simulink library "sm_wheel_loader_lib"  (R2025a)
settings: Solver=VariableStepAuto  StartTime=0.0  StopTime=10.0  RelTol=1e-3
undefined symbols (not defined in the file): AToTOrificeVector, BiPOrificeVector, boomHEArea, boomREArea, BToTOrificeVector, fluids, GRake, GToothL, GToothR, HMPST, HydFcnParams, logLoad, Position, PToAOrificeVector, PToBOrificeVector, RakeL, RakeR, testInput, Wheel_Loader, X, Y, Z
libraries: sm_lib x694, fl_lib x183, nesl_utility x74, SimscapeFluids_lib x62, sdl_lib x25, cvt_components_lib x25, simulink_extras x5, $bdroot x4, wheel_loader_contact_lib x4, ee_lib x2, SignalEditorBlockLib x1, batteryecm_lib x1
(part 21 of 26)

== system sm_wheel_loader_lib/Wheel Loader Vehicle/Driveline/Driveline/Driveline 3D/Differential F/Stub Shaft R ==
  FDRStubShaft_primary : sm_lib/Body Elements/File Solid  ExtGeomFileName=DiffF_Stub_Shaft_R.STEP  UnitType=FromFile  ExtGeomFileUnits=m  StepReaderType=HEX  ExportConvexHullGeometry=off  InertiaType=Custom  BasedOnType=DensityFromFile  Density=1000  DensityUnits=kg/m^3  Mass=Wheel_Loader.bodyGroups(43).subGroups(1).inertialProperties.mass  MassUnits=kg  CenterOfMass="Wheel_Loader.bodyGroups(43).subGroups(1).inertialProperties.centerOfMass-[0 -0.000000705905842  -0.000000386215069]'"  CenterOfMassUnits=m  MomentsOfInertia=Wheel_Loader.bodyGroups(43).subGroups(1).inertialProperties.momentsOfInertia  MomentsOfInertiaUnits=kg*m^2  ProductsOfInertia=Wheel_Loader.bodyGroups(43).subGroups(1).inertialProperties.productsOfInertia  ProductsOfInertiaUnits=kg*m^2  GraphicType=FromGeometry  MarkerShape=Sphere  MarkerSize=10  GraphicVisPropType=SimpleVisualProperties  GraphicDiffuseColor=Wheel_Loader.bodyGroups(43).subGroups(1).visualProperties.rgb  GraphicOpacity=Wheel_Loader.bodyGroups(43).subGroups(1).visualProperties.opacity  GraphicSpecularColor=[0.5 0.5 0.5 1.0]  GraphicAmbientColor=[0.15 0.15 0.15 1.0]  GraphicEmissiveColor=[0.0 0.0 0.0 1.0]  GraphicShininess=75  DoExposeReferenceFrame=on  SerializedFrames=<Frames/>
  FDRStubShaft_secondary : sm_lib/Body Elements/File Solid  ExtGeomFileName=DiffF_Stub_Shaft_R_Spacer.STEP  UnitType=FromFile  ExtGeomFileUnits=m  StepReaderType=HEX  ExportConvexHullGeometry=off  InertiaType=Custom  BasedOnType=DensityFromFile  Density=1000  DensityUnits=kg/m^3  Mass=Wheel_Loader.bodyGroups(43).subGroups(2).inertialProperties.mass  MassUnits=kg  CenterOfMass="Wheel_Loader.bodyGroups(43).subGroups(2).inertialProperties.centerOfMass-[0 -0.000000705905966  -0.000000386213852]'"  CenterOfMassUnits=m  MomentsOfInertia=Wheel_Loader.bodyGroups(43).subGroups(2).inertialProperties.momentsOfInertia  MomentsOfInertiaUnits=kg*m^2  ProductsOfInertia=Wheel_Loader.bodyGroups(43).subGroups(2).inertialProperties.productsOfInertia  ProductsOfInertiaUnits=kg*m^2  GraphicType=FromGeometry  MarkerShape=Sphere  MarkerSize=10  GraphicVisPropType=SimpleVisualProperties  GraphicDiffuseColor=Wheel_Loader.bodyGroups(43).subGroups(2).visualProperties.rgb  GraphicOpacity=Wheel_Loader.bodyGroups(43).subGroups(2).visualProperties.opacity  GraphicSpecularColor=[0.5 0.5 0.5 1.0]  GraphicAmbientColor=[0.15 0.15 0.15 1.0]  GraphicEmissiveColor=[0.0 0.0 0.0 1.0]  GraphicShininess=75  DoExposeReferenceFrame=on  SerializedFrames=<Frames/>
  RT_FDRStubShaft_RFFDSunGear_Weld : sm_lib/Frames and Transforms/Rigid Transform  RotationMethod=RotationMatrix  FollAlignAxisA=+X  BaseAlignAxisA=+Y  FollAlignAxisB=+Y  BaseAlignAxisB=+Z  RotationStandardAxis=+Z  RotationAngle=0.0  RotationAngleUnits=deg  RotationArbitraryAxis=[0 0 1]  RotationSequenceAxes=FollowerAxes  RotationSequence=XYX  RotationSequenceAngles=[0 0 0]  RotationSequenceAnglesUnits=deg  RotationMatrix=Wheel_Loader.coordSys(66).transform.rotation  Quaternion=[1 0 0 0]  TranslationMethod=Cartesian  TranslationCartesianOffset=Wheel_Loader.coordSys(66).transform.translation  TranslationCartesianOffsetUnits=m  TranslationStandardAxis=+Z  TranslationStandardOffset=0  TranslationStandardOffsetUnits=m  TranslationROffset=0  TranslationROffsetUnits=m  TranslationThetaOffset=0  TranslationThetaOffsetUnits=deg  TranslationZOffset=0  TranslationZOffsetUnits=m
  RT_FDR_StubShaft_Casing : sm_lib/Frames and Transforms/Rigid Transform  RotationMethod=RotationMatrix  FollAlignAxisA=+X  BaseAlignAxisA=+Y  FollAlignAxisB=+Y  BaseAlignAxisB=+Z  RotationStandardAxis=+Z  RotationAngle=0.0  RotationAngleUnits=deg  RotationArbitraryAxis=[0 0 1]  RotationSequenceAxes=FollowerAxes  RotationSequence=XYX  RotationSequenceAngles=[0 0 0]  RotationSequenceAnglesUnits=deg  RotationMatrix=Wheel_Loader.coordSys(49).transform.rotation  Quaternion=[1 0 0 0]  TranslationMethod=Cartesian  TranslationCartesianOffset=Wheel_Loader.coordSys(49).transform.translation  TranslationCartesianOffsetUnits=m  TranslationStandardAxis=+Z  TranslationStandardOffset=0  TranslationStandardOffsetUnits=m  TranslationROffset=0  TranslationROffsetUnits=m  TranslationThetaOffset=0  TranslationThetaOffsetUnits=deg  TranslationZOffset=0  TranslationZOffsetUnits=m
  RT_FDR_StubShaft_SideGear : sm_lib/Frames and Transforms/Rigid Transform  RotationMethod=RotationMatrix  FollAlignAxisA=+X  BaseAlignAxisA=+Y  FollAlignAxisB=+Y  BaseAlignAxisB=+Z  RotationStandardAxis=+Z  RotationAngle=0.0  RotationAngleUnits=deg  RotationArbitraryAxis=[0 0 1]  RotationSequenceAxes=FollowerAxes  RotationSequence=XYX  RotationSequenceAngles=[0 0 0]  RotationSequenceAnglesUnits=deg  RotationMatrix=Wheel_Loader.coordSys(49).transform.rotation  Quaternion=[1 0 0 0]  TranslationMethod=Cartesian  TranslationCartesianOffset=Wheel_Loader.coordSys(49).transform.translation  TranslationCartesianOffsetUnits=m  TranslationStandardAxis=+Z  TranslationStandardOffset=0  TranslationStandardOffsetUnits=m  TranslationROffset=0  TranslationROffsetUnits=m  TranslationThetaOffset=0  TranslationThetaOffsetUnits=deg  TranslationZOffset=0  TranslationZOffsetUnits=m
  RT_FrontAxle_FDRStubShaft : sm_lib/Frames and Transforms/Rigid Transform  RotationMethod=RotationMatrix  FollAlignAxisA=+X  BaseAlignAxisA=+Y  FollAlignAxisB=+Y  BaseAlignAxisB=+Z  RotationStandardAxis=+Z  RotationAngle=0.0  RotationAngleUnits=deg  RotationArbitraryAxis=[0 0 1]  RotationSequenceAxes=FollowerAxes  RotationSequence=XYX  RotationSequenceAngles=[0 0 0]  RotationSequenceAnglesUnits=deg  RotationMatrix=Wheel_Loader.coordSys(49).transform.rotation  Quaternion=[1 0 0 0]  TranslationMethod=Cartesian  TranslationCartesianOffset=Wheel_Loader.coordSys(49).transform.translation  TranslationCartesianOffsetUnits=m  TranslationStandardAxis=+Z  TranslationStandardOffset=0  TranslationStandardOffsetUnits=m  TranslationROffset=0  TranslationROffsetUnits=m  TranslationThetaOffset=0  TranslationThetaOffsetUnits=deg  TranslationZOffset=0  TranslationZOffsetUnits=m
  F3 : PMIOPort  Side=Left
  F1 : PMIOPort  Port=2  Side=Right
  connections:
  RT_FDRStubShaft_RFFDSunGear_Weld/RConn1 -- F3/RConn1
  RT_FDR_StubShaft_SideGear/RConn1 -- F1/RConn1
  RT_FDR_StubShaft_SideGear/LConn1 -- RT_FrontAxle_FDRStubShaft/LConn1 -- FDRStubShaft_secondary/RConn1 -- FDRStubShaft_primary/RConn1 -- RT_FDRStubShaft_RFFDSunGear_Weld/LConn1 -- RT_FDR_StubShaft_Casing/LConn1

== system sm_wheel_loader_lib/Wheel Loader Vehicle/Driveline/Driveline/Driveline 3D/Differential R/Ring Gear ==
  Casing A : sm_lib/Body Elements/File Solid  ExtGeomFileName=DiffR_Casing_A.STEP  UnitType=FromFile  ExtGeomFileUnits=m  StepReaderType=HEX  ExportConvexHullGeometry=off  InertiaType=Custom  BasedOnType=DensityFromFile  Density=1000  DensityUnits=kg/m^3  Mass=Wheel_Loader.bodyGroups(69).subGroups(1).inertialProperties.mass  MassUnits=kg  CenterOfMass=Wheel_Loader.bodyGroups(69).subGroups(1).inertialProperties.centerOfMass  CenterOfMassUnits=m  MomentsOfInertia=Wheel_Loader.bodyGroups(69).subGroups(1).inertialProperties.momentsOfInertia  MomentsOfInertiaUnits=kg*m^2  ProductsOfInertia=Wheel_Loader.bodyGroups(69).subGroups(1).inertialProperties.productsOfInertia  ProductsOfInertiaUnits=kg*m^2  GraphicType=FromGeometry  MarkerShape=Sphere  MarkerSize=10  GraphicVisPropType=SimpleVisualProperties  GraphicDiffuseColor=Wheel_Loader.bodyGroups(69).subGroups(1).visualProperties.rgb  GraphicOpacity=diffR_casing_opc  GraphicSpecularColor=[0.5 0.5 0.5 1.0]  GraphicAmbientColor=[0.15 0.15 0.15 1.0]  GraphicEmissiveColor=[0.0 0.0 0.0 1.0]  GraphicShininess=75  DoExposeReferenceFrame=on  SerializedFrames=<Frames/>
  Casing B : sm_lib/Body Elements/File Solid  ExtGeomFileName=DiffR_Casing_B.STEP  UnitType=FromFile  ExtGeomFileUnits=m  StepReaderType=HEX  ExportConvexHullGeometry=off  InertiaType=Custom  BasedOnType=DensityFromFile  Density=1000  DensityUnits=kg/m^3  Mass=Wheel_Loader.bodyGroups(69).subGroups(2).inertialProperties.mass  MassUnits=kg  CenterOfMass=Wheel_Loader.bodyGroups(69).subGroups(2).inertialProperties.centerOfMass  CenterOfMassUnits=m  MomentsOfInertia=Wheel_Loader.bodyGroups(69).subGroups(2).inertialProperties.momentsOfInertia  MomentsOfInertiaUnits=kg*m^2  ProductsOfInertia=Wheel_Loader.bodyGroups(69).subGroups(2).inertialProperties.productsOfInertia  ProductsOfInertiaUnits=kg*m^2  GraphicType=FromGeometry  MarkerShape=Sphere  MarkerSize=10  GraphicVisPropType=SimpleVisualProperties  GraphicDiffuseColor=Wheel_Loader.bodyGroups(69).subGroups(2).visualProperties.rgb  GraphicOpacity=diffR_casing_opc  GraphicSpecularColor=[0.5 0.5 0.5 1.0]  GraphicAmbientColor=[0.15 0.15 0.15 1.0]  GraphicEmissiveColor=[0.0 0.0 0.0 1.0]  GraphicShininess=75  DoExposeReferenceFrame=on  SerializedFrames=<Frames/>
  RT_RDL_StubShaft_Casing : sm_lib/Frames and Transforms/Rigid Transform  RotationMethod=RotationMatrix  FollAlignAxisA=+X  BaseAlignAxisA=+Y  FollAlignAxisB=+Y  BaseAlignAxisB=+Z  RotationStandardAxis=+Z  RotationAngle=0.0  RotationAngleUnits=deg  RotationArbitraryAxis=[0 0 1]  RotationSequenceAxes=FollowerAxes  RotationSequence=XYX  RotationSequenceAngles=[0 0 0]  RotationSequenceAnglesUnits=deg  RotationMatrix=Wheel_Loader.coordSys(48).transform.rotation  Quaternion=[1 0 0 0]  TranslationMethod=Cartesian  TranslationCartesianOffset=Wheel_Loader.coordSys(48).transform.translation  TranslationCartesianOffsetUnits=m  TranslationStandardAxis=+Z  TranslationStandardOffset=0  TranslationStandardOffsetUnits=m  TranslationROffset=0  TranslationROffsetUnits=m  TranslationThetaOffset=0  TranslationThetaOffsetUnits=deg  TranslationZOffset=0  TranslationZOffsetUnits=m
  RT_RD_Pinion_Ring_BGC : sm_lib/Frames and Transforms/Rigid Transform  RotationMethod=RotationMatrix  FollAlignAxisA=+X  BaseAlignAxisA=+Y  FollAlignAxisB=+Y  BaseAlignAxisB=+Z  RotationStandardAxis=+Z  RotationAngle=0.0  RotationAngleUnits=deg  RotationArbitraryAxis=[0 0 1]  RotationSequenceAxes=FollowerAxes  RotationSequence=XYX  RotationSequenceAngles=[0 0 0]  RotationSequenceAnglesUnits=deg  RotationMatrix=Wheel_Loader.coordSys(47).transform.rotation  Quaternion=[1 0 0 0]  TranslationMethod=Cartesian  TranslationCartesianOffset=Wheel_Loader.coordSys(47).transform.translation  TranslationCartesianOffsetUnits=m  TranslationStandardAxis=+Z  TranslationStandardOffset=0  TranslationStandardOffsetUnits=m  TranslationROffset=0  TranslationROffsetUnits=m  TranslationThetaOffset=0  TranslationThetaOffsetUnits=deg  TranslationZOffset=0  TranslationZOffsetUnits=m
  Ring Gear : sm_lib/Body Elements/File Solid  ExtGeomFileName=DiffR_Ring_Gear.STEP  UnitType=FromFile  ExtGeomFileUnits=m  StepReaderType=HEX  ExportConvexHullGeometry=off  InertiaType=Custom  BasedOnType=DensityFromFile  Density=1000  DensityUnits=kg/m^3  Mass=Wheel_Loader.bodyGroups(65).subGroups(1).inertialProperties.mass  MassUnits=kg  CenterOfMass=Wheel_Loader.bodyGroups(65).subGroups(1).inertialProperties.centerOfMass  CenterOfMassUnits=m  MomentsOfInertia=Wheel_Loader.bodyGroups(65).subGroups(1).inertialProperties.momentsOfInertia  MomentsOfInertiaUnits=kg*m^2  ProductsOfInertia=Wheel_Loader.bodyGroups(65).subGroups(1).inertialProperties.productsOfInertia  ProductsOfInertiaUnits=kg*m^2  GraphicType=FromGeometry  MarkerShape=Sphere  MarkerSize=10  GraphicVisPropType=SimpleVisualProperties  GraphicDiffuseColor=Wheel_Loader.bodyGroups(65).subGroups(1).visualProperties.rgb  GraphicOpacity=Wheel_Loader.bodyGroups(65).subGroups(1).visualProperties.opacity  GraphicSpecularColor=[0.5 0.5 0.5 1.0]  GraphicAmbientColor=[0.15 0.15 0.15 1.0]  GraphicEmissiveColor=[0.0 0.0 0.0 1.0]  GraphicShininess=75  DoExposeReferenceFrame=on  SerializedFrames=<Frames/>
  Transform CG : sm_lib/Frames and Transforms/Rigid Transform  RotationMethod=None  FollAlignAxisA=+X  BaseAlignAxisA=+Y  FollAlignAxisB=+Y  BaseAlignAxisB=+Z  RotationStandardAxis=+Z  RotationAngle=0.0  RotationAngleUnits=deg  RotationArbitraryAxis=[0 0 1]  RotationSequenceAxes=FollowerAxes  RotationSequence=XYX  RotationSequenceAngles=[0 0 0]  RotationSequenceAnglesUnits=deg  RotationMatrix=[1 0 0; 0 1 0; 0 0 1]  Quaternion=[1 0 0 0]  TranslationMethod=Cartesian  TranslationCartesianOffset=[0 -0.000000002038373 0.000000042999574]  TranslationCartesianOffsetUnits=m  TranslationStandardAxis=+Z  TranslationStandardOffset=0  TranslationStandardOffsetUnits=m  TranslationROffset=0  TranslationROffsetUnits=m  TranslationThetaOffset=0  TranslationThetaOffsetUnits=deg  TranslationZOffset=0  TranslationZOffsetUnits=m
  Transform Side Gear L : sm_lib/Frames and Transforms/Rigid Transform  RotationMethod=StandardAxis  FollAlignAxisA=+X  BaseAlignAxisA=+Y  FollAlignAxisB=+Y  BaseAlignAxisB=+Z  RotationStandardAxis=+Y  RotationAngle=-90  RotationAngleUnits=deg  RotationArbitraryAxis=[0 0 1]  RotationSequenceAxes=FollowerAxes  RotationSequence=XYX  RotationSequenceAngles=[0 0 0]  RotationSequenceAnglesUnits=deg  RotationMatrix=[1 0 0; 0 1 0; 0 0 1]  Quaternion=[1 0 0 0]  TranslationMethod=Cartesian  TranslationCartesianOffset=[0.056 0 0.0896 ]/2  TranslationCartesianOffsetUnits=m  TranslationStandardAxis=+Z  TranslationStandardOffset=0  TranslationStandardOffsetUnits=m  TranslationROffset=0  TranslationROffsetUnits=m  TranslationThetaOffset=0  TranslationThetaOffsetUnits=deg  TranslationZOffset=0  TranslationZOffsetUnits=m
  Transform Spider Gear 2 : sm_lib/Frames and Transforms/Rigid Transform  RotationMethod=StandardAxis  FollAlignAxisA=+X  BaseAlignAxisA=+Y  FollAlignAxisB=+Y  BaseAlignAxisB=+Z  RotationStandardAxis=+Y  RotationAngle=-90  RotationAngleUnits=deg  RotationArbitraryAxis=[0 0 1]  RotationSequenceAxes=FollowerAxes  RotationSequence=XYX  RotationSequenceAngles=[0 0 0]  RotationSequenceAnglesUnits=deg  RotationMatrix=[1 0 0; 0 1 0; 0 0 1]  Quaternion=[1 0 0 0]  TranslationMethod=Cartesian  TranslationCartesianOffset=[0.0896 0 0.056]/2  TranslationCartesianOffsetUnits=m  TranslationStandardAxis=+Z  TranslationStandardOffset=0  TranslationStandardOffsetUnits=m  TranslationROffset=0  TranslationROffsetUnits=m  TranslationThetaOffset=0  TranslationThetaOffsetUnits=deg  TranslationZOffset=0  TranslationZOffsetUnits=m
  Pin : PMIOPort  Side=Left
  SGR : PMIOPort  Port=2  Side=Right
  connections:
  RT_RD_Pinion_Ring_BGC/LConn1 -- Ring Gear/RConn1 -- RT_RDL_StubShaft_Casing/LConn1 -- Transform CG/LConn1
  RT_RDL_StubShaft_Casing/RConn1 -- Transform Spider Gear 2/LConn1
  RT_RD_Pinion_Ring_BGC/RConn1 -- Pin/RConn1
  Transform CG/RConn1 -- Casing A/RConn1 -- Casing B/RConn1
  Transform Spider Gear 2/RConn1 -- Transform Side Gear L/LConn1
  SGR/RConn1 -- Transform Side Gear L/RConn1

== system sm_wheel_loader_lib/Wheel Loader Vehicle/Driveline/Driveline/Driveline 3D/Differential R/Side Gear L ==
  RT_RDL_StubShaft_SideGear : sm_lib/Frames and Transforms/Rigid Transform  RotationMethod=RotationMatrix  FollAlignAxisA=+X  BaseAlignAxisA=+Y  FollAlignAxisB=+Y  BaseAlignAxisB=+Z  RotationStandardAxis=+Z  RotationAngle=0.0  RotationAngleUnits=deg  RotationArbitraryAxis=[0 0 1]  RotationSequenceAxes=FollowerAxes  RotationSequence=XYX  RotationSequenceAngles=[0 0 0]  RotationSequenceAnglesUnits=deg  RotationMatrix=Wheel_Loader.coordSys(48).transform.rotation  Quaternion=[1 0 0 0]  TranslationMethod=Cartesian  TranslationCartesianOffset=Wheel_Loader.coordSys(48).transform.translation  TranslationCartesianOffsetUnits=m  TranslationStandardAxis=+Z  TranslationStandardOffset=0  TranslationStandardOffsetUnits=m  TranslationROffset=0  TranslationROffsetUnits=m  TranslationThetaOffset=0  TranslationThetaOffsetUnits=deg  TranslationZOffset=0  TranslationZOffsetUnits=m
  RT_RDSpiderGear1_RDLSideGear_BGC : sm_lib/Frames and Transforms/Rigid Transform  RotationMethod=RotationMatrix  FollAlignAxisA=+X  BaseAlignAxisA=+Y  FollAlignAxisB=+Y  BaseAlignAxisB=+Z  RotationStandardAxis=+Z  RotationAngle=0.0  RotationAngleUnits=deg  RotationArbitraryAxis=[0 0 1]  RotationSequenceAxes=FollowerAxes  RotationSequence=XYX  RotationSequenceAngles=[0 0 0]  RotationSequenceAnglesUnits=deg  RotationMatrix=Wheel_Loader.coordSys(48).transform.rotation  Quaternion=[1 0 0 0]  TranslationMethod=Cartesian  TranslationCartesianOffset=Wheel_Loader.coordSys(48).transform.translation  TranslationCartesianOffsetUnits=m  TranslationStandardAxis=+Z  TranslationStandardOffset=0  TranslationStandardOffsetUnits=m  TranslationROffset=0  TranslationROffsetUnits=m  TranslationThetaOffset=0  TranslationThetaOffsetUnits=deg  TranslationZOffset=0  TranslationZOffsetUnits=m
  RT_RDSpiderGear2_RDLSideGear_BGC : sm_lib/Frames and Transforms/Rigid Transform  RotationMethod=RotationMatrix  FollAlignAxisA=+X  BaseAlignAxisA=+Y  FollAlignAxisB=+Y  BaseAlignAxisB=+Z  RotationStandardAxis=+Z  RotationAngle=0.0  RotationAngleUnits=deg  RotationArbitraryAxis=[0 0 1]  RotationSequenceAxes=FollowerAxes  RotationSequence=XYX  RotationSequenceAngles=[0 0 0]  RotationSequenceAnglesUnits=deg  RotationMatrix=Wheel_Loader.coordSys(48).transform.rotation  Quaternion=[1 0 0 0]  TranslationMethod=Cartesian  TranslationCartesianOffset=Wheel_Loader.coordSys(48).transform.translation  TranslationCartesianOffsetUnits=m  TranslationStandardAxis=+Z  TranslationStandardOffset=0  TranslationStandardOffsetUnits=m  TranslationROffset=0  TranslationROffsetUnits=m  TranslationThetaOffset=0  TranslationThetaOffsetUnits=deg  TranslationZOffset=0  TranslationZOffsetUnits=m
  Side Gear L : sm_lib/Body Elements/File Solid  ExtGeomFileName=DiffR_Side_Gear_L.STEP  UnitType=FromFile  ExtGeomFileUnits=m  StepReaderType=HEX  ExportConvexHullGeometry=off  InertiaType=Custom  BasedOnType=DensityFromFile  Density=1000  DensityUnits=kg/m^3  Mass=Wheel_Loader.bodyGroups(57).subGroups(1).inertialProperties.mass  MassUnits=kg  CenterOfMass=Wheel_Loader.bodyGroups(57).subGroups(1).inertialProperties.centerOfMass  CenterOfMassUnits=m  MomentsOfInertia=Wheel_Loader.bodyGroups(57).subGroups(1).inertialProperties.momentsOfInertia  MomentsOfInertiaUnits=kg*m^2  ProductsOfInertia=Wheel_Loader.bodyGroups(57).subGroups(1).inertialProperties.productsOfInertia  ProductsOfInertiaUnits=kg*m^2  GraphicType=FromGeometry  MarkerShape=Sphere  MarkerSize=10  GraphicVisPropType=SimpleVisualProperties  GraphicDiffuseColor=Wheel_Loader.bodyGroups(57).subGroups(1).visualProperties.rgb  GraphicOpacity=Wheel_Loader.bodyGroups(57).subGroups(1).visualProperties.opacity  GraphicSpecularColor=[0.5 0.5 0.5 1.0]  GraphicAmbientColor=[0.15 0.15 0.15 1.0]  GraphicEmissiveColor=[0.0 0.0 0.0 1.0]  GraphicShininess=75  DoExposeReferenceFrame=on  SerializedFrames=<Frames/>
  B : PMIOPort  Side=Left
  F : PMIOPort  Port=2  Side=Right
  connections:
  B/RConn1 -- RT_RDL_StubShaft_SideGear/RConn1 -- F/RConn1
  RT_RDSpiderGear2_RDLSideGear_BGC/LConn1 -- RT_RDSpiderGear1_RDLSideGear_BGC/LConn1 -- Side Gear L/RConn1 -- RT_RDL_StubShaft_SideGear/LConn1

== system sm_wheel_loader_lib/Wheel Loader Vehicle/Driveline/Driveline/Driveline 3D/Differential R/Side Gear R ==
  RT_RDSpiderGear1toRDRSideGear_BGC : sm_lib/Frames and Transforms/Rigid Transform  RotationMethod=RotationMatrix  FollAlignAxisA=+X  BaseAlignAxisA=+Y  FollAlignAxisB=+Y  BaseAlignAxisB=+Z  RotationStandardAxis=+Z  RotationAngle=0.0  RotationAngleUnits=deg  RotationArbitraryAxis=[0 0 1]  RotationSequenceAxes=FollowerAxes  RotationSequence=XYX  RotationSequenceAngles=[0 0 0]  RotationSequenceAnglesUnits=deg  RotationMatrix=Wheel_Loader.coordSys(52).transform.rotation  Quaternion=[1 0 0 0]  TranslationMethod=Cartesian  TranslationCartesianOffset=Wheel_Loader.coordSys(52).transform.translation  TranslationCartesianOffsetUnits=m  TranslationStandardAxis=+Z  TranslationStandardOffset=0  TranslationStandardOffsetUnits=m  TranslationROffset=0  TranslationROffsetUnits=m  TranslationThetaOffset=0  TranslationThetaOffsetUnits=deg  TranslationZOffset=0  TranslationZOffsetUnits=m
  Side Gear R : sm_lib/Body Elements/File Solid  ExtGeomFileName=DiffR_Side_Gear_R.STEP  UnitType=FromFile  ExtGeomFileUnits=m  StepReaderType=HEX  ExportConvexHullGeometry=off  InertiaType=Custom  BasedOnType=DensityFromFile  Density=1000  DensityUnits=kg/m^3  Mass=Wheel_Loader.bodyGroups(56).subGroups(1).inertialProperties.mass  MassUnits=kg  CenterOfMass=Wheel_Loader.bodyGroups(56).subGroups(1).inertialProperties.centerOfMass  CenterOfMassUnits=m  MomentsOfInertia=Wheel_Loader.bodyGroups(56).subGroups(1).inertialProperties.momentsOfInertia  MomentsOfInertiaUnits=kg*m^2  ProductsOfInertia=Wheel_Loader.bodyGroups(56).subGroups(1).inertialProperties.productsOfInertia  ProductsOfInertiaUnits=kg*m^2  GraphicType=FromGeometry  MarkerShape=Sphere  MarkerSize=10  GraphicVisPropType=SimpleVisualProperties  GraphicDiffuseColor=Wheel_Loader.bodyGroups(56).subGroups(1).visualProperties.rgb  GraphicOpacity=Wheel_Loader.bodyGroups(56).subGroups(1).visualProperties.opacity  GraphicSpecularColor=[0.5 0.5 0.5 1.0]  GraphicAmbientColor=[0.15 0.15 0.15 1.0]  GraphicEmissiveColor=[0.0 0.0 0.0 1.0]  GraphicShininess=75  DoExposeReferenceFrame=on  SerializedFrames=<Frames/>
  B : PMIOPort  Side=Left
  F : PMIOPort  Port=2  Side=Right
  connections:
  Side Gear R/RConn1 -- RT_RDSpiderGear1toRDRSideGear_BGC/LConn1
  B/RConn1 -- RT_RDSpiderGear1toRDRSideGear_BGC/RConn1 -- F/RConn1

== system sm_wheel_loader_lib/Wheel Loader Vehicle/Driveline/Driveline/Driveline 3D/Differential R/Spider Gear 1 ==
  Gear : sm_lib/Body Elements/File Solid  ExtGeomFileName=DiffR_Spider_Gear1.STEP  UnitType=FromFile  ExtGeomFileUnits=m  StepReaderType=HEX  ExportConvexHullGeometry=off  InertiaType=Custom  BasedOnType=DensityFromFile  Density=1000  DensityUnits=kg/m^3  Mass=Wheel_Loader.bodyGroups(61).subGroups(1).inertialProperties.mass  MassUnits=kg  CenterOfMass=Wheel_Loader.bodyGroups(61).subGroups(1).inertialProperties.centerOfMass  CenterOfMassUnits=m  MomentsOfInertia=Wheel_Loader.bodyGroups(61).subGroups(1).inertialProperties.momentsOfInertia  MomentsOfInertiaUnits=kg*m^2  ProductsOfInertia=Wheel_Loader.bodyGroups(61).subGroups(1).inertialProperties.productsOfInertia  ProductsOfInertiaUnits=kg*m^2  GraphicType=FromGeometry  MarkerShape=Sphere  MarkerSize=10  GraphicVisPropType=SimpleVisualProperties  GraphicDiffuseColor=Wheel_Loader.bodyGroups(61).subGroups(1).visualProperties.rgb  GraphicOpacity=Wheel_Loader.bodyGroups(61).subGroups(1).visualProperties.opacity  GraphicSpecularColor=[0.5 0.5 0.5 1.0]  GraphicAmbientColor=[0.15 0.15 0.15 1.0]  GraphicEmissiveColor=[0.0 0.0 0.0 1.0]  GraphicShininess=75  DoExposeReferenceFrame=on  SerializedFrames=<Frames/>
  RT_RDSpiderGear1_RDLSideGear_BGC : sm_lib/Frames and Transforms/Rigid Transform  RotationMethod=RotationMatrix  FollAlignAxisA=+X  BaseAlignAxisA=+Y  FollAlignAxisB=+Y  BaseAlignAxisB=+Z  RotationStandardAxis=+Z  RotationAngle=0.0  RotationAngleUnits=deg  RotationArbitraryAxis=[0 0 1]  RotationSequenceAxes=FollowerAxes  RotationSequence=XYX  RotationSequenceAngles=[0 0 0]  RotationSequenceAnglesUnits=deg  RotationMatrix=Wheel_Loader.coordSys(54).transform.rotation  Quaternion=[1 0 0 0]  TranslationMethod=Cartesian  TranslationCartesianOffset=Wheel_Loader.coordSys(54).transform.translation  TranslationCartesianOffsetUnits=m  TranslationStandardAxis=+Z  TranslationStandardOffset=0  TranslationStandardOffsetUnits=m  TranslationROffset=0  TranslationROffsetUnits=m  TranslationThetaOffset=0  TranslationThetaOffsetUnits=deg  TranslationZOffset=0  TranslationZOffsetUnits=m
  RT_RDSpiderGear1toRDRSideGear_BGC : sm_lib/Frames and Transforms/Rigid Transform  RotationMethod=RotationMatrix  FollAlignAxisA=+X  BaseAlignAxisA=+Y  FollAlignAxisB=+Y  BaseAlignAxisB=+Z  RotationStandardAxis=+Z  RotationAngle=0.0  RotationAngleUnits=deg  RotationArbitraryAxis=[0 0 1]  RotationSequenceAxes=FollowerAxes  RotationSequence=XYX  RotationSequenceAngles=[0 0 0]  RotationSequenceAnglesUnits=deg  RotationMatrix=Wheel_Loader.coordSys(54).transform.rotation  Quaternion=[1 0 0 0]  TranslationMethod=Cartesian  TranslationCartesianOffset=Wheel_Loader.coordSys(54).transform.translation  TranslationCartesianOffsetUnits=m  TranslationStandardAxis=+Z  TranslationStandardOffset=0  TranslationStandardOffsetUnits=m  TranslationROffset=0  TranslationROffsetUnits=m  TranslationThetaOffset=0  TranslationThetaOffsetUnits=deg  TranslationZOffset=0  TranslationZOffsetUnits=m
  RT_RD_Casing_SpiderGear1 : sm_lib/Frames and Transforms/Rigid Transform  RotationMethod=RotationMatrix  FollAlignAxisA=+X  BaseAlignAxisA=+Y  FollAlignAxisB=+Y  BaseAlignAxisB=+Z  RotationStandardAxis=+Z  RotationAngle=0.0  RotationAngleUnits=deg  RotationArbitraryAxis=[0 0 1]  RotationSequenceAxes=FollowerAxes  RotationSequence=XYX  RotationSequenceAngles=[0 0 0]  RotationSequenceAnglesUnits=deg  RotationMatrix=Wheel_Loader.coordSys(54).transform.rotation  Quaternion=[1 0 0 0]  TranslationMethod=Cartesian  TranslationCartesianOffset=Wheel_Loader.coordSys(54).transform.translation  TranslationCartesianOffsetUnits=m  TranslationStandardAxis=+Z  TranslationStandardOffset=0  TranslationStandardOffsetUnits=m  TranslationROffset=0  TranslationROffsetUnits=m  TranslationThetaOffset=0  TranslationThetaOffsetUnits=deg  TranslationZOffset=0  TranslationZOffsetUnits=m
  Shaft : sm_lib/Body Elements/File Solid  ExtGeomFileName=DiffR_Spider_Gear1_Shaft.STEP  UnitType=FromFile  ExtGeomFileUnits=m  StepReaderType=HEX  ExportConvexHullGeometry=off  InertiaType=Custom  BasedOnType=DensityFromFile  Density=1000  DensityUnits=kg/m^3  Mass=Wheel_Loader.bodyGroups(61).subGroups(2).inertialProperties.mass  MassUnits=kg  CenterOfMass=Wheel_Loader.bodyGroups(61).subGroups(2).inertialProperties.centerOfMass  CenterOfMassUnits=m  MomentsOfInertia=Wheel_Loader.bodyGroups(61).subGroups(2).inertialProperties.momentsOfInertia  MomentsOfInertiaUnits=kg*m^2  ProductsOfInertia=Wheel_Loader.bodyGroups(61).subGroups(2).inertialProperties.productsOfInertia  ProductsOfInertiaUnits=kg*m^2  GraphicType=FromGeometry  MarkerShape=Sphere  MarkerSize=10  GraphicVisPropType=SimpleVisualProperties  GraphicDiffuseColor=Wheel_Loader.bodyGroups(61).subGroups(2).visualProperties.rgb  GraphicOpacity=Wheel_Loader.bodyGroups(61).subGroups(2).visualProperties.opacity  GraphicSpecularColor=[0.5 0.5 0.5 1.0]  GraphicAmbientColor=[0.15 0.15 0.15 1.0]  GraphicEmissiveColor=[0.0 0.0 0.0 1.0]  GraphicShininess=75  DoExposeReferenceFrame=on  SerializedFrames=<Frames/>
  B : PMIOPort  Side=Left
  F : PMIOPort  Port=2  Side=Right
  connections:
  B/RConn1 -- RT_RD_Casing_SpiderGear1/RConn1 -- F/RConn1
  RT_RD_Casing_SpiderGear1/LConn1 -- Shaft/RConn1 -- Gear/RConn1 -- RT_RDSpiderGear1toRDRSideGear_BGC/LConn1 -- RT_RDSpiderGear1_RDLSideGear_BGC/LConn1

== system sm_wheel_loader_lib/Wheel Loader Vehicle/Driveline/Driveline/Driveline 3D/Differential R/Spider Gear 2 ==
  Gear : sm_lib/Body Elements/File Solid  ExtGeomFileName=DiffR_Spider_Gear2.STEP  UnitType=FromFile  ExtGeomFileUnits=m  StepReaderType=HEX  ExportConvexHullGeometry=off  InertiaType=Custom  BasedOnType=DensityFromFile  Density=1000  DensityUnits=kg/m^3  Mass=Wheel_Loader.bodyGroups(67).subGroups(1).inertialProperties.mass  MassUnits=kg  CenterOfMass=Wheel_Loader.bodyGroups(67).subGroups(1).inertialProperties.centerOfMass  CenterOfMassUnits=m  MomentsOfInertia=Wheel_Loader.bodyGroups(67).subGroups(1).inertialProperties.momentsOfInertia  MomentsOfInertiaUnits=kg*m^2  ProductsOfInertia=Wheel_Loader.bodyGroups(67).subGroups(1).inertialProperties.productsOfInertia  ProductsOfInertiaUnits=kg*m^2  GraphicType=FromGeometry  MarkerShape=Sphere  MarkerSize=10  GraphicVisPropType=SimpleVisualProperties  GraphicDiffuseColor=Wheel_Loader.bodyGroups(67).subGroups(1).visualProperties.rgb  GraphicOpacity=Wheel_Loader.bodyGroups(67).subGroups(1).visualProperties.opacity  GraphicSpecularColor=[0.5 0.5 0.5 1.0]  GraphicAmbientColor=[0.15 0.15 0.15 1.0]  GraphicEmissiveColor=[0.0 0.0 0.0 1.0]  GraphicShininess=75  DoExposeReferenceFrame=on  SerializedFrames=<Frames/>
  RT_RDSpiderGear2_RDLSideGear_BGC : sm_lib/Frames and Transforms/Rigid Transform  RotationMethod=RotationMatrix  FollAlignAxisA=+X  BaseAlignAxisA=+Y  FollAlignAxisB=+Y  BaseAlignAxisB=+Z  RotationStandardAxis=+Z  RotationAngle=0.0  RotationAngleUnits=deg  RotationArbitraryAxis=[0 0 1]  RotationSequenceAxes=FollowerAxes  RotationSequence=XYX  RotationSequenceAngles=[0 0 0]  RotationSequenceAnglesUnits=deg  RotationMatrix=Wheel_Loader.coordSys(50).transform.rotation  Quaternion=[1 0 0 0]  TranslationMethod=Cartesian  TranslationCartesianOffset=Wheel_Loader.coordSys(50).transform.translation  TranslationCartesianOffsetUnits=m  TranslationStandardAxis=+Z  TranslationStandardOffset=0  TranslationStandardOffsetUnits=m  TranslationROffset=0  TranslationROffsetUnits=m  TranslationThetaOffset=0  TranslationThetaOffsetUnits=deg  TranslationZOffset=0  TranslationZOffsetUnits=m
  RT_RDSpiderGear2_RDRSideGear_BGC : sm_lib/Frames and Transforms/Rigid Transform  RotationMethod=RotationMatrix  FollAlignAxisA=+X  BaseAlignAxisA=+Y  FollAlignAxisB=+Y  BaseAlignAxisB=+Z  RotationStandardAxis=+Z  RotationAngle=0.0  RotationAngleUnits=deg  RotationArbitraryAxis=[0 0 1]  RotationSequenceAxes=FollowerAxes  RotationSequence=XYX  RotationSequenceAngles=[0 0 0]  RotationSequenceAnglesUnits=deg  RotationMatrix=Wheel_Loader.coordSys(50).transform.rotation  Quaternion=[1 0 0 0]  TranslationMethod=Cartesian  TranslationCartesianOffset=Wheel_Loader.coordSys(50).transform.translation  TranslationCartesianOffsetUnits=m  TranslationStandardAxis=+Z  TranslationStandardOffset=0  TranslationStandardOffsetUnits=m  TranslationROffset=0  TranslationROffsetUnits=m  TranslationThetaOffset=0  TranslationThetaOffsetUnits=deg  TranslationZOffset=0  TranslationZOffsetUnits=m
  RT_RD_Casing_SpiderGear2 : sm_lib/Frames and Transforms/Rigid Transform  RotationMethod=RotationMatrix  FollAlignAxisA=+X  BaseAlignAxisA=+Y  FollAlignAxisB=+Y  BaseAlignAxisB=+Z  RotationStandardAxis=+Z  RotationAngle=0.0  RotationAngleUnits=deg  RotationArbitraryAxis=[0 0 1]  RotationSequenceAxes=FollowerAxes  RotationSequence=XYX  RotationSequenceAngles=[0 0 0]  RotationSequenceAnglesUnits=deg  RotationMatrix=Wheel_Loader.coordSys(50).transform.rotation  Quaternion=[1 0 0 0]  TranslationMethod=Cartesian  TranslationCartesianOffset=Wheel_Loader.coordSys(50).transform.translation  TranslationCartesianOffsetUnits=m  TranslationStandardAxis=+Z  TranslationStandardOffset=0  TranslationStandardOffsetUnits=m  TranslationROffset=0  TranslationROffsetUnits=m  TranslationThetaOffset=0  TranslationThetaOffsetUnits=deg  TranslationZOffset=0  TranslationZOffsetUnits=m
  Shaft : sm_lib/Body Elements/File Solid  ExtGeomFileName=DiffR_Spider_Gear2_Shaft.STEP  UnitType=FromFile  ExtGeomFileUnits=m  StepReaderType=HEX  ExportConvexHullGeometry=off  InertiaType=Custom  BasedOnType=DensityFromFile  Density=1000  DensityUnits=kg/m^3  Mass=Wheel_Loader.bodyGroups(67).subGroups(2).inertialProperties.mass  MassUnits=kg  CenterOfMass=Wheel_Loader.bodyGroups(67).subGroups(2).inertialProperties.centerOfMass  CenterOfMassUnits=m  MomentsOfInertia=Wheel_Loader.bodyGroups(67).subGroups(2).inertialProperties.momentsOfInertia  MomentsOfInertiaUnits=kg*m^2  ProductsOfInertia=Wheel_Loader.bodyGroups(67).subGroups(2).inertialProperties.productsOfInertia  ProductsOfInertiaUnits=kg*m^2  GraphicType=FromGeometry  MarkerShape=Sphere  MarkerSize=10  GraphicVisPropType=SimpleVisualProperties  GraphicDiffuseColor=Wheel_Loader.bodyGroups(67).subGroups(2).visualProperties.rgb  GraphicOpacity=Wheel_Loader.bodyGroups(67).subGroups(2).visualProperties.opacity  GraphicSpecularColor=[0.5 0.5 0.5 1.0]  GraphicAmbientColor=[0.15 0.15 0.15 1.0]  GraphicEmissiveColor=[0.0 0.0 0.0 1.0]  GraphicShininess=75  DoExposeReferenceFrame=on  SerializedFrames=<Frames/>
  B : PMIOPort  Side=Left
  F : PMIOPort  Port=2  Side=Right
  connections:
  B/RConn1 -- RT_RD_Casing_SpiderGear2/RConn1 -- F/RConn1
  RT_RDSpiderGear2_RDRSideGear_BGC/LConn1 -- RT_RDSpiderGear2_RDLSideGear_BGC/LConn1 -- Shaft/RConn1 -- Gear/RConn1 -- RT_RD_Casing_SpiderGear2/LConn1

== system sm_wheel_loader_lib/Wheel Loader Vehicle/Driveline/Driveline/Driveline 3D/Differential R/Stub Shaft L ==
  RT_RDLStubShaft_LRFDSunGear_Weld : sm_lib/Frames and Transforms/Rigid Transform  RotationMethod=RotationMatrix  FollAlignAxisA=+X  BaseAlignAxisA=+Y  FollAlignAxisB=+Y  BaseAlignAxisB=+Z  RotationStandardAxis=+Z  RotationAngle=0.0  RotationAngleUnits=deg  RotationArbitraryAxis=[0 0 1]  RotationSequenceAxes=FollowerAxes  RotationSequence=XYX  RotationSequenceAngles=[0 0 0]  RotationSequenceAnglesUnits=deg  RotationMatrix=Wheel_Loader.coordSys(62).transform.rotation  Quaternion=[1 0 0 0]  TranslationMethod=Cartesian  TranslationCartesianOffset=Wheel_Loader.coordSys(62).transform.translation  TranslationCartesianOffsetUnits=m  TranslationStandardAxis=+Z  TranslationStandardOffset=0  TranslationStandardOffsetUnits=m  TranslationROffset=0  TranslationROffsetUnits=m  TranslationThetaOffset=0  TranslationThetaOffsetUnits=deg  TranslationZOffset=0  TranslationZOffsetUnits=m
  RT_RDL_StubShaft_Casing : sm_lib/Frames and Transforms/Rigid Transform  RotationMethod=RotationMatrix  FollAlignAxisA=+X  BaseAlignAxisA=+Y  FollAlignAxisB=+Y  BaseAlignAxisB=+Z  RotationStandardAxis=+Z  RotationAngle=0.0  RotationAngleUnits=deg  RotationArbitraryAxis=[0 0 1]  RotationSequenceAxes=FollowerAxes  RotationSequence=XYX  RotationSequenceAngles=[0 0 0]  RotationSequenceAnglesUnits=deg  RotationMatrix=Wheel_Loader.coordSys(48).transform.rotation  Quaternion=[1 0 0 0]  TranslationMethod=Cartesian  TranslationCartesianOffset=Wheel_Loader.coordSys(48).transform.translation  TranslationCartesianOffsetUnits=m  TranslationStandardAxis=+Z  TranslationStandardOffset=0  TranslationStandardOffsetUnits=m  TranslationROffset=0  TranslationROffsetUnits=m  TranslationThetaOffset=0  TranslationThetaOffsetUnits=deg  TranslationZOffset=0  TranslationZOffsetUnits=m
  Shaft : sm_lib/Body Elements/File Solid  ExtGeomFileName=DiffR_Stub_Shaft_L.STEP  UnitType=FromFile  ExtGeomFileUnits=m  StepReaderType=HEX  ExportConvexHullGeometry=off  InertiaType=Custom  BasedOnType=DensityFromFile  Density=1000  DensityUnits=kg/m^3  Mass=Wheel_Loader.bodyGroups(47).subGroups(1).inertialProperties.mass  MassUnits=kg  CenterOfMass=Wheel_Loader.bodyGroups(47).subGroups(1).inertialProperties.centerOfMass+[0 0.000000714421034 0.000000370227091]'  CenterOfMassUnits=m  MomentsOfInertia=Wheel_Loader.bodyGroups(47).subGroups(1).inertialProperties.momentsOfInertia  MomentsOfInertiaUnits=kg*m^2  ProductsOfInertia=Wheel_Loader.bodyGroups(47).subGroups(1).inertialProperties.productsOfInertia  ProductsOfInertiaUnits=kg*m^2  GraphicType=FromGeometry  MarkerShape=Sphere  MarkerSize=10  GraphicVisPropType=SimpleVisualProperties  GraphicDiffuseColor=Wheel_Loader.bodyGroups(47).subGroups(1).visualProperties.rgb  GraphicOpacity=Wheel_Loader.bodyGroups(47).subGroups(1).visualProperties.opacity  GraphicSpecularColor=[0.5 0.5 0.5 1.0]  GraphicAmbientColor=[0.15 0.15 0.15 1.0]  GraphicEmissiveColor=[0.0 0.0 0.0 1.0]  GraphicShininess=75  DoExposeReferenceFrame=on  SerializedFrames=<Frames/>
  Spacer : sm_lib/Body Elements/File Solid  ExtGeomFileName=DiffR_Stub_Shaft_L_Spacer.STEP  UnitType=FromFile  ExtGeomFileUnits=m  StepReaderType=HEX  ExportConvexHullGeometry=off  InertiaType=Custom  BasedOnType=DensityFromFile  Density=1000  DensityUnits=kg/m^3  Mass=Wheel_Loader.bodyGroups(47).subGroups(2).inertialProperties.mass  MassUnits=kg  CenterOfMass=Wheel_Loader.bodyGroups(47).subGroups(2).inertialProperties.centerOfMass+[0 0.000000714419972 0.000000370227621]'  CenterOfMassUnits=m  MomentsOfInertia=Wheel_Loader.bodyGroups(47).subGroups(2).inertialProperties.momentsOfInertia  MomentsOfInertiaUnits=kg*m^2  ProductsOfInertia=Wheel_Loader.bodyGroups(47).subGroups(2).inertialProperties.productsOfInertia  ProductsOfInertiaUnits=kg*m^2  GraphicType=FromGeometry  MarkerShape=Sphere  MarkerSize=10  GraphicVisPropType=SimpleVisualProperties  GraphicDiffuseColor=Wheel_Loader.bodyGroups(47).subGroups(2).visualProperties.rgb  GraphicOpacity=Wheel_Loader.bodyGroups(47).subGroups(2).visualProperties.opacity  GraphicSpecularColor=[0.5 0.5 0.5 1.0]  GraphicAmbientColor=[0.15 0.15 0.15 1.0]  GraphicEmissiveColor=[0.0 0.0 0.0 1.0]  GraphicShininess=75  DoExposeReferenceFrame=on  SerializedFrames=<Frames/>
  Transform Frame Offset : sm_lib/Frames and Transforms/Rigid Transform  RotationMethod=None  FollAlignAxisA=+X  BaseAlignAxisA=+Y  FollAlignAxisB=+Y  BaseAlignAxisB=+Z  RotationStandardAxis=+Z  RotationAngle=0.0  RotationAngleUnits=deg  RotationArbitraryAxis=[0 0 1]  RotationSequenceAxes=FollowerAxes  RotationSequence=XYX  RotationSequenceAngles=[0 0 0]  RotationSequenceAnglesUnits=deg  RotationMatrix=[1 0 0; 0 1 0; 0 0 1]  Quaternion=[1 0 0 0]  TranslationMethod=Cartesian  TranslationCartesianOffset="-[-0.000000000000120   0.000000000000452 0]"  TranslationCartesianOffsetUnits=m  TranslationStandardAxis=+Z  TranslationStandardOffset=0  TranslationStandardOffsetUnits=m  TranslationROffset=0  TranslationROffsetUnits=m  TranslationThetaOffset=0  TranslationThetaOffsetUnits=deg  TranslationZOffset=0  TranslationZOffsetUnits=m
  F2 : PMIOPort  Side=Right
  F3 : PMIOPort  Port=2  Side=Left
  connections:
  RT_RDLStubShaft_LRFDSunGear_Weld/RConn1 -- F3/RConn1
  Transform Frame Offset/LConn1 -- RT_RDL_StubShaft_Casing/RConn1
  RT_RDLStubShaft_LRFDSunGear_Weld/LConn1 -- RT_RDL_StubShaft_Casing/LConn1 -- Shaft/RConn1 -- Spacer/RConn1
  Transform Frame Offset/RConn1 -- F2/RConn1

== system sm_wheel_loader_lib/Wheel Loader Vehicle/Driveline/Driveline/Driveline 3D/Differential R/Stub Shaft R ==
  RT_RDRStubShaft_RRFDSunGear_Weld : sm_lib/Frames and Transforms/Rigid Transform  RotationMethod=RotationMatrix  FollAlignAxisA=+X  BaseAlignAxisA=+Y  FollAlignAxisB=+Y  BaseAlignAxisB=+Z  RotationStandardAxis=+Z  RotationAngle=0.0  RotationAngleUnits=deg  RotationArbitraryAxis=[0 0 1]  RotationSequenceAxes=FollowerAxes  RotationSequence=XYX  RotationSequenceAngles=[0 0 0]  RotationSequenceAnglesUnits=deg  RotationMatrix=Wheel_Loader.coordSys(58).transform.rotation  Quaternion=[1 0 0 0]  TranslationMethod=Cartesian  TranslationCartesianOffset=Wheel_Loader.coordSys(58).transform.translation  TranslationCartesianOffsetUnits=m  TranslationStandardAxis=+Z  TranslationStandardOffset=0  TranslationStandardOffsetUnits=m  TranslationROffset=0  TranslationROffsetUnits=m  TranslationThetaOffset=0  TranslationThetaOffsetUnits=deg  TranslationZOffset=0  TranslationZOffsetUnits=m
  RT_RDR_StubShaft_SideGear : sm_lib/Frames and Transforms/Rigid Transform  RotationMethod=RotationMatrix  FollAlignAxisA=+X  BaseAlignAxisA=+Y  FollAlignAxisB=+Y  BaseAlignAxisB=+Z  RotationStandardAxis=+Z  RotationAngle=0.0  RotationAngleUnits=deg  RotationArbitraryAxis=[0 0 1]  RotationSequenceAxes=FollowerAxes  RotationSequence=XYX  RotationSequenceAngles=[0 0 0]  RotationSequenceAnglesUnits=deg  RotationMatrix=Wheel_Loader.coordSys(52).transform.rotation  Quaternion=[1 0 0 0]  TranslationMethod=Cartesian  TranslationCartesianOffset=Wheel_Loader.coordSys(52).transform.translation  TranslationCartesianOffsetUnits=m  TranslationStandardAxis=+Z  TranslationStandardOffset=0  TranslationStandardOffsetUnits=m  TranslationROffset=0  TranslationROffsetUnits=m  TranslationThetaOffset=0  TranslationThetaOffsetUnits=deg  TranslationZOffset=0  TranslationZOffsetUnits=m
  Shaft : sm_lib/Body Elements/File Solid  ExtGeomFileName=DiffR_Stub_Shaft_R.STEP  UnitType=FromFile  ExtGeomFileUnits=m  StepReaderType=HEX  ExportConvexHullGeometry=off  InertiaType=Custom  BasedOnType=DensityFromFile  Density=1000  DensityUnits=kg/m^3  Mass=Wheel_Loader.bodyGroups(46).subGroups(1).inertialProperties.mass  MassUnits=kg  CenterOfMass=Wheel_Loader.bodyGroups(46).subGroups(1).inertialProperties.centerOfMass  CenterOfMassUnits=m  MomentsOfInertia=Wheel_Loader.bodyGroups(46).subGroups(1).inertialProperties.momentsOfInertia  MomentsOfInertiaUnits=kg*m^2  ProductsOfInertia=Wheel_Loader.bodyGroups(46).subGroups(1).inertialProperties.productsOfInertia  ProductsOfInertiaUnits=kg*m^2  GraphicType=FromGeometry  MarkerShape=Sphere  MarkerSize=10  GraphicVisPropType=SimpleVisualProperties  GraphicDiffuseColor=Wheel_Loader.bodyGroups(46).subGroups(1).visualProperties.rgb  GraphicOpacity=Wheel_Loader.bodyGroups(46).subGroups(1).visualProperties.opacity  GraphicSpecularColor=[0.5 0.5 0.5 1.0]  GraphicAmbientColor=[0.15 0.15 0.15 1.0]  GraphicEmissiveColor=[0.0 0.0 0.0 1.0]  GraphicShininess=75  DoExposeReferenceFrame=on  SerializedFrames=<Frames/>
  Spacer : sm_lib/Body Elements/File Solid  ExtGeomFileName=DiffR_Stub_Shaft_R_Spacer.STEP  UnitType=FromFile  ExtGeomFileUnits=m  StepReaderType=HEX  ExportConvexHullGeometry=off  InertiaType=Custom  BasedOnType=DensityFromFile  Density=1000  DensityUnits=kg/m^3  Mass=Wheel_Loader.bodyGroups(46).subGroups(2).inertialProperties.mass  MassUnits=kg  CenterOfMass=Wheel_Loader.bodyGroups(46).subGroups(2).inertialProperties.centerOfMass  CenterOfMassUnits=m  MomentsOfInertia=Wheel_Loader.bodyGroups(46).subGroups(2).inertialProperties.momentsOfInertia  MomentsOfInertiaUnits=kg*m^2  ProductsOfInertia=Wheel_Loader.bodyGroups(46).subGroups(2).inertialProperties.productsOfInertia  ProductsOfInertiaUnits=kg*m^2  GraphicType=FromGeometry  MarkerShape=Sphere  MarkerSize=10  GraphicVisPropType=SimpleVisualProperties  GraphicDiffuseColor=Wheel_Loader.bodyGroups(46).subGroups(2).visualProperties.rgb  GraphicOpacity=Wheel_Loader.bodyGroups(46).subGroups(2).visualProperties.opacity  GraphicSpecularColor=[0.5 0.5 0.5 1.0]  GraphicAmbientColor=[0.15 0.15 0.15 1.0]  GraphicEmissiveColor=[0.0 0.0 0.0 1.0]  GraphicShininess=75  DoExposeReferenceFrame=on  SerializedFrames=<Frames/>
  F : PMIOPort  Side=Right
  B : PMIOPort  Port=2  Side=Left
  connections:
  Shaft/RConn1 -- Spacer/RConn1 -- RT_RDRStubShaft_RRFDSunGear_Weld/LConn1 -- RT_RDR_StubShaft_SideGear/LConn1
  RT_RDRStubShaft_RRFDSunGear_Weld/RConn1 -- F/RConn1
  B/RConn1 -- RT_RDR_StubShaft_SideGear/RConn1

== system sm_wheel_loader_lib/Wheel Loader Vehicle/Driveline/Driveline/Driveline 3D/Driveshaft Front/FrontAxleUJoint ==
  Pinion_Spacer : sm_lib/Body Elements/File Solid  ExtGeomFileName=DiffF_Pinion_Spacer.STEP  UnitType=FromFile  ExtGeomFileUnits=m  StepReaderType=HEX  ExportConvexHullGeometry=off  InertiaType=Custom  BasedOnType=DensityFromFile  Density=1000  DensityUnits=kg/m^3  Mass=Wheel_Loader.bodyGroups(48).subGroups(2).inertialProperties.mass  MassUnits=kg  CenterOfMass=Wheel_Loader.bodyGroups(48).subGroups(2).inertialProperties.centerOfMass  CenterOfMassUnits=m  MomentsOfInertia=Wheel_Loader.bodyGroups(48).subGroups(2).inertialProperties.momentsOfInertia  MomentsOfInertiaUnits=kg*m^2  ProductsOfInertia=Wheel_Loader.bodyGroups(48).subGroups(2).inertialProperties.productsOfInertia  ProductsOfInertiaUnits=kg*m^2  GraphicType=FromGeometry  MarkerShape=Sphere  MarkerSize=10  GraphicVisPropType=SimpleVisualProperties  GraphicDiffuseColor=Wheel_Loader.bodyGroups(48).subGroups(2).visualProperties.rgb  GraphicOpacity=Wheel_Loader.bodyGroups(48).subGroups(2).visualProperties.opacity  GraphicSpecularColor=[0.5 0.5 0.5 1.0]  GraphicAmbientColor=[0.15 0.15 0.15 1.0]  GraphicEmissiveColor=[0.0 0.0 0.0 1.0]  GraphicShininess=75  DoExposeReferenceFrame=on  SerializedFrames=<Frames/>
  RT_FDPinion_FrontAxleUjoint : sm_lib/Frames and Transforms/Rigid Transform  RotationMethod=RotationMatrix  FollAlignAxisA=+X  BaseAlignAxisA=+Y  FollAlignAxisB=+Y  BaseAlignAxisB=+Z  RotationStandardAxis=+Z  RotationAngle=0.0  RotationAngleUnits=deg  RotationArbitraryAxis=[0 0 1]  RotationSequenceAxes=FollowerAxes  RotationSequence=XYX  RotationSequenceAngles=[0 0 0]  RotationSequenceAnglesUnits=deg  RotationMatrix=Wheel_Loader.coordSys(44).transform.rotation  Quaternion=[1 0 0 0]  TranslationMethod=Cartesian  TranslationCartesianOffset=Wheel_Loader.coordSys(44).transform.translation  TranslationCartesianOffsetUnits=m  TranslationStandardAxis=+Z  TranslationStandardOffset=0  TranslationStandardOffsetUnits=m  TranslationROffset=0  TranslationROffsetUnits=m  TranslationThetaOffset=0  TranslationThetaOffsetUnits=deg  TranslationZOffset=0  TranslationZOffsetUnits=m
  RT_FDPinion_FrontAxleUjoint1 : sm_lib/Frames and Transforms/Rigid Transform  RotationMethod=RotationMatrix  FollAlignAxisA=+X  BaseAlignAxisA=+Y  FollAlignAxisB=+Y  BaseAlignAxisB=+Z  RotationStandardAxis=+Z  RotationAngle=0.0  RotationAngleUnits=deg  RotationArbitraryAxis=[0 0 1]  RotationSequenceAxes=FollowerAxes  RotationSequence=XYX  RotationSequenceAngles=[0 0 0]  RotationSequenceAnglesUnits=deg  RotationMatrix=Wheel_Loader.coordSys(44).transform.rotation  Quaternion=[1 0 0 0]  TranslationMethod=Cartesian  TranslationCartesianOffset=Wheel_Loader.coordSys(44).transform.translation  TranslationCartesianOffsetUnits=m  TranslationStandardAxis=+Z  TranslationStandardOffset=0  TranslationStandardOffsetUnits=m  TranslationROffset=0  TranslationROffsetUnits=m  TranslationThetaOffset=0  TranslationThetaOffsetUnits=deg  TranslationZOffset=0  TranslationZOffsetUnits=m
  X : PMIOPort  Side=Left
  A : PMIOPort  Port=2  Side=Right
  connections:
  RT_FDPinion_FrontAxleUjoint/RConn1 -- RT_FDPinion_FrontAxleUjoint1/RConn1
  RT_FDPinion_FrontAxleUjoint1/LConn1 -- X/RConn1 -- Pinion_Spacer/RConn1
  RT_FDPinion_FrontAxleUjoint/LConn1 -- A/RConn1

== system sm_wheel_loader_lib/Wheel Loader Vehicle/Driveline/Driveline/Driveline 3D/Driveshaft Front/Intermediate Shaft ==
  Intermediate_ShaftF : sm_lib/Body Elements/File Solid  ExtGeomFileName=Driveline_Intermediate_ShaftF.STEP  UnitType=FromFile  ExtGeomFileUnits=m  StepReaderType=HEX  ExportConvexHullGeometry=off  InertiaType=Custom  BasedOnType=DensityFromFile  Density=1000  DensityUnits=kg/m^3  Mass=Wheel_Loader.bodyGroups(38).subGroups(1).inertialProperties.mass  MassUnits=kg  CenterOfMass=Wheel_Loader.bodyGroups(38).subGroups(1).inertialProperties.centerOfMass  CenterOfMassUnits=m  MomentsOfInertia=Wheel_Loader.bodyGroups(38).subGroups(1).inertialProperties.momentsOfInertia  MomentsOfInertiaUnits=kg*m^2  ProductsOfInertia=Wheel_Loader.bodyGroups(38).subGroups(1).inertialProperties.productsOfInertia  ProductsOfInertiaUnits=kg*m^2  GraphicType=FromGeometry  MarkerShape=Sphere  MarkerSize=10  GraphicVisPropType=SimpleVisualProperties  GraphicDiffuseColor=Wheel_Loader.bodyGroups(38).subGroups(1).visualProperties.rgb  GraphicOpacity=Wheel_Loader.bodyGroups(38).subGroups(1).visualProperties.opacity  GraphicSpecularColor=[0.5 0.5 0.5 1.0]  GraphicAmbientColor=[0.15 0.15 0.15 1.0]  GraphicEmissiveColor=[0.0 0.0 0.0 1.0]  GraphicShininess=75  DoExposeReferenceFrame=on  SerializedFrames=<Frames/>
  RT_FrontDriveShaft_MidShipShaft : sm_lib/Frames and Transforms/Rigid Transform  RotationMethod=RotationMatrix  FollAlignAxisA=+X  BaseAlignAxisA=+Y  FollAlignAxisB=+Y  BaseAlignAxisB=+Z  RotationStandardAxis=+Z  RotationAngle=0.0  RotationAngleUnits=deg  RotationArbitraryAxis=[0 0 1]  RotationSequenceAxes=FollowerAxes  RotationSequence=XYX  RotationSequenceAngles=[0 0 0]  RotationSequenceAnglesUnits=deg  RotationMatrix=Wheel_Loader.coordSys(22).transform.rotation  Quaternion=[1 0 0 0]  TranslationMethod=Cartesian  TranslationCartesianOffset=Wheel_Loader.coordSys(22).transform.translation  TranslationCartesianOffsetUnits=m  TranslationStandardAxis=+Z  TranslationStandardOffset=0  TranslationStandardOffsetUnits=m  TranslationROffset=0  TranslationROffsetUnits=m  TranslationThetaOffset=0  TranslationThetaOffsetUnits=deg  TranslationZOffset=0  TranslationZOffsetUnits=m
  F1 : PMIOPort  Side=Right
  B2 : PMIOPort  Port=2  Side=Left
  connections:
  RT_FrontDriveShaft_MidShipShaft/RConn1 -- F1/RConn1
  RT_FrontDriveShaft_MidShipShaft/LConn1 -- B2/RConn1 -- Intermediate_ShaftF/RConn1

== system sm_wheel_loader_lib/Wheel Loader Vehicle/Driveline/Driveline/Driveline 3D/Driveshaft Front/Joint ==
  CV Joint : Subsystem  VariantControl=CV_Joint
      mask Display: image('sm_wheel_loader_driveline_cvjointF_IMAGE.png');
  U Joint : Subsystem  VariantControl=U_Joint
      mask Display: image('sm_wheel_loader_driveline_ujointF_IMAGE.png');
  B : PMIOPort  Side=Left
  F : PMIOPort  Port=2  Side=Right
